simulink model "PI_control"  (R2026a)
settings: Solver=VariableStepAuto  StopTime=3
undefined symbols (not defined in the file): K, Kp, sigma
libraries: simulink x2, slpidlib x1
settings Model: Creator=nateg  LastModifiedBy=nateg

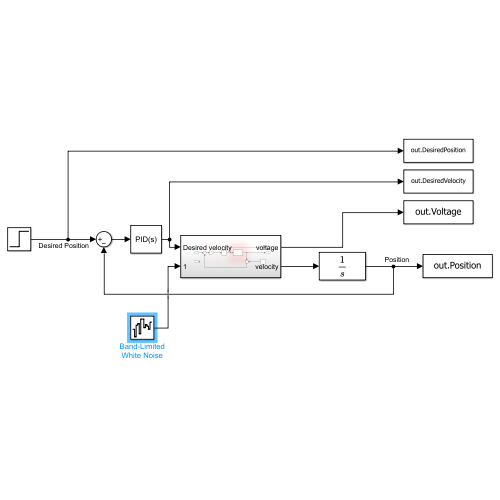
[thumbnail: Simulink's stored preview of the top-level diagram]
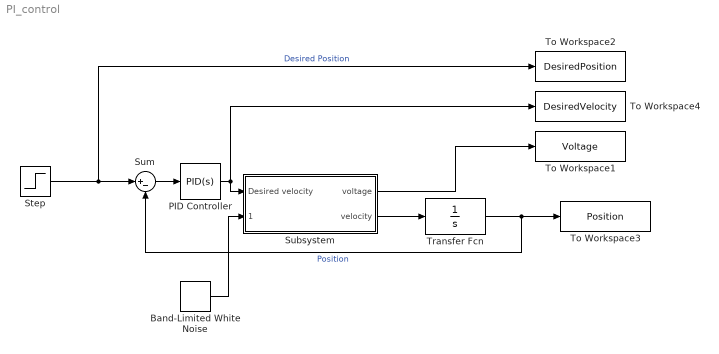
== system PI_control ==
  Band-Limited White Noise : simulink/Sources/Band-Limited White Noise  Cov=[0.001]  Ts=0.01  seed=[23341]
  PID Controller : slpidlib/PID Controller  Controller=PID  Form=Parallel  TimeDomain=Continuous-time  UseExternalTs=off  SampleTime=-1  IntegratorMethod=Forward Euler  FilterMethod=Forward Euler  ControllerParametersSource=internal  P=1  I=1  UseKiTs=off  D=0  UseExternalDerivativeSource=off  N=100  UseFilter=on  TunerSelectOption=Transfer Function Based (PID Tuner App)  InitialConditionSource=internal  InitialConditionForIntegrator=0  InitialConditionForFilter=0  DifferentiatorICPrevScaledInput=0  ExternalReset=none  TrackingMode=off  Kt=1  LimitOutput=off  SatLimitsSource=internal  UpperSaturationLimit=inf  LowerSaturationLimit=-inf  LinearizeAsGain=on  AntiWindupMode=none  Kb=1  LimitIntegrator=off  UpperIntegratorSaturationLimit=inf  LowerIntegratorSaturationLimit=-inf  POutMin=[]  POutMax=[]  IOutMin=[]  IOutMax=[]  DOutMin=[]  DOutMax=[]  NOutMin=[]  NOutMax=[]  SumOutMin=[]  SumOutMax=[]  SaturationOutMin=[]  SaturationOutMax=[]  PParamMin=[]  PParamMax=[]  IParamMin=[]  IParamMax=[]  DParamMin=[]  DParamMax=[]  NParamMin=[]  NParamMax=[]  KbParamMin=[]  KbParamMax=[]  KtParamMin=[]  KtParamMax=[]  KbOutMin=[]  KbOutMax=[]  KtOutMin=[]  KtOutMax=[]  IntegratorOutMin=[]  IntegratorOutMax=[]  FilterOutMin=[]  FilterOutMax=[]  SumI1OutMin=[]  SumI1OutMax=[]  SumI2OutMin=[]  SumI2OutMax=[]  SumI3OutMin=[]  SumI3OutMax=[]  SumI4OutMin=[]  SumI4OutMax=[]  SumDOutMin=[]  SumDOutMax=[]  DifferentiatorOutMin=[]  DifferentiatorOutMax=[]  FilterDiffOutCoefMin=[]  FilterDiffOutCoefMax=[]  ReciprocalOutMin=[]  ReciprocalOutMax=[]  SumDenOutMin=[]  SumDenOutMax=[]  SumNumOutMin=[]  SumNumOutMax=[]  DivideOutMin=[]  DivideOutMax=[]  UdiffTsProdOutMin=[]  UdiffTsProdOutMax=[]  NTsProdOutMin=[]  NTsProdOutMax=[]  UintegralTsProdOutMin=[]  UintegralTsProdOutMax=[]  UngainTsProdOutMin=[]  UngainTsProdOutMax=[]  ClampingZeroOutDataTypeStr=Inherit: Inherit via back propagation  ClampingZeroOutMin=[]  ClampingZeroOutMax=[]  FilterDenConstantOutDataTypeStr=Inherit: Inherit via back propagation  FilterDenConstantOutMin=[]  FilterDenConstantOutMax=[]  PCopyOutDataTypeStr=Inherit: Inherit via back propagation  PCopyOutMin=[]  PCopyOutMax=[]  NCopyOutDataTypeStr=Inherit: Inherit via back propagation  NCopyOutMin=[]  NCopyOutMax=[]  IntegratorContinuousStateAttributes=''  IntegratorStateMustResolveToSignalObject=off  IntegratorRTWStateStorageClass=Auto  FilterContinuousStateAttributes=''  FilterStateMustResolveToSignalObject=off  FilterRTWStateStorageClass=Auto  ParallelPVariant=InternalParameters  IdealPVariant=Disabled  IVariant=InternalParameters  DVariant=InternalParameters  IntegratorVariant=Continuous  SatVariant=Disabled  AWVariant=Passthrough  PCopyVariant=Disabled  TRVariant=Disabled  FdbkBlocksVariant=Forward  IdealPFdbkVariant=Disabled  SatFdbkVariant=Disabled  DerivativeFilterVariant=ContFilter  NVariant=InternalParameters  NCopyVariant=Disabled  FilterICVariant=InternalICsFilter  IntegratorICVariant=InternalICs  ExternalResetVariant=Disabled  TRSumVariant=Passthrough  SumFdbkVariant=Disabled  SumVariant=Sum_PID  TsampFilterVariant=InternalTs  TsampNgainVariant=Passthrough  TsampIntegralVariant=Disabled_SignalSpec  ExternalSaturationOutDataTypeStr=Inherit: Same as second input  DerivativeSourceVariant=ErrorSignal  PreIntVariant=InternalPreInt
  Step : Step  FinalValue=3.14159  SampleTime=0
  Subsystem : Subsystem
  Sum : Sum  Inputs=|+-
  To Workspace1 : ToWorkspace  VariableName=Voltage  SaveFormat=Timeseries  SampleTime=-1
  To Workspace2 : ToWorkspace  VariableName=DesiredPosition  SaveFormat=Timeseries  SampleTime=-1
  To Workspace3 : ToWorkspace  VariableName=Position  SaveFormat=Timeseries  SampleTime=-1
  To Workspace4 : ToWorkspace  VariableName=DesiredVelocity  SaveFormat=Timeseries  SampleTime=-1
  Transfer Fcn : TransferFcn  Denominator=[1 0]
  wires:
  Step/1 -> Sum/1, To Workspace2/1  "Desired Position"
  Subsystem/2(velocity) -> Transfer Fcn/1
  Transfer Fcn/1 -> Sum/2, To Workspace3/1  "Position"
  Sum/1 -> PID Controller/1
  PID Controller/1 -> To Workspace4/1, Subsystem/1(Desired velocity)
  Band-Limited White Noise/1 -> Subsystem/2(1)
  Subsystem/1(voltage) -> To Workspace1/1

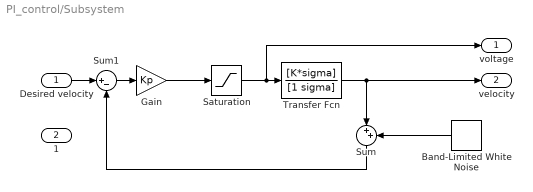
== system PI_control/Subsystem ==
  Desired velocity : Inport
  1 : Inport  Port=2
  Band-Limited White Noise : simulink/Sources/Band-Limited White Noise  Cov=[0.0001]  Ts=0.01  seed=[23341]
  Gain : Gain  Gain=Kp
  Saturation : Saturate  UpperLimit=7.5
  Sum : Sum  Inputs=|++
  Sum1 : Sum  Inputs=|+-
  Transfer Fcn : TransferFcn  Numerator=[K*sigma]  Denominator=[1 sigma]
  voltage : Outport
  velocity : Outport  Port=2
  wires:
  Gain/1 -> Saturation/1
  Band-Limited White Noise/1 -> Sum/2
  Transfer Fcn/1 -> velocity/1, Sum/1
  Sum/1 -> Sum1/2
  Saturation/1 -> voltage/1, Transfer Fcn/1
  Sum1/1 -> Gain/1
  Desired velocity/1 -> Sum1/1
